simulink model "HaulagePhysicsKinematicsBridge"  (R2026a)
settings: Solver=ode23t  StopTime=390  MaxStep=0.05
PostLoadFcn:
  | stage12ModelFile = get_param(bdroot, 'FileName');
  | stage12ProjectRoot = fileparts(fileparts(stage12ModelFile));
  | addpath(stage12ProjectRoot);
  | loadStage12PhysicsKinematicsBridgeInputs(stage12ProjectRoot);
  | clear stage12ModelFile stage12ProjectRoot
InitFcn:
  | stage12ModelFile = get_param(bdroot, 'FileName');
  | stage12ProjectRoot = fileparts(fileparts(stage12ModelFile));
  | addpath(stage12ProjectRoot);
  | loadStage12PhysicsKinematicsBridgeInputs(stage12ProjectRoot);
  | clear stage12ModelFile stage12ProjectRoot
libraries: nesl_utility x6, fl_lib x3, sdl_lib x1, robotmobilelib x1
settings Model: Creator=chimb  LastModifiedBy=chimb

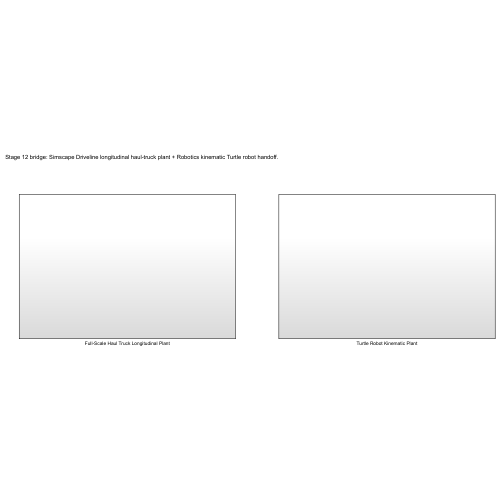
[thumbnail: Simulink's stored preview of the top-level diagram]
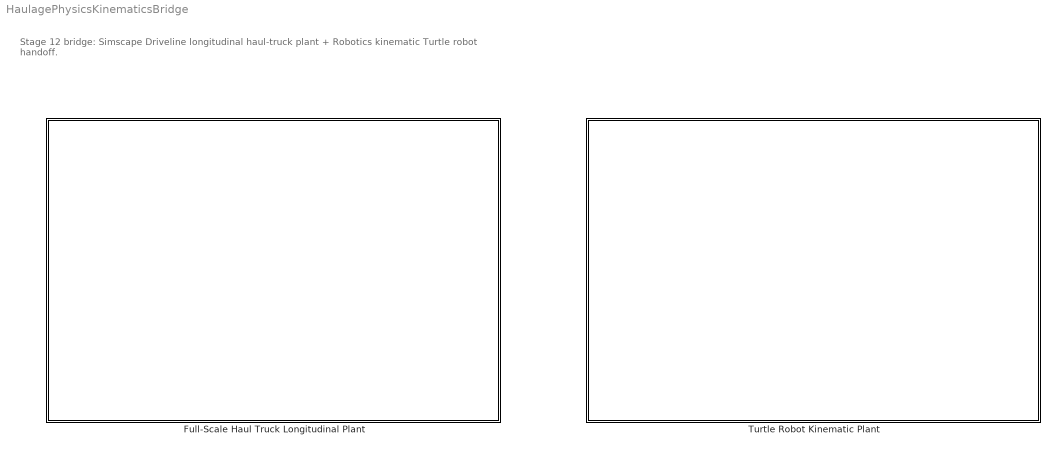
== system HaulagePhysicsKinematicsBridge ==
  note: Stage 12 bridge: Simscape Driveline longitudinal haul-truck plant + Robotics kinematic Turtle robot handoff.
  Full-Scale Haul Truck Longitudinal Plant : Subsystem
  Turtle Robot Kinematic Plant : Subsystem

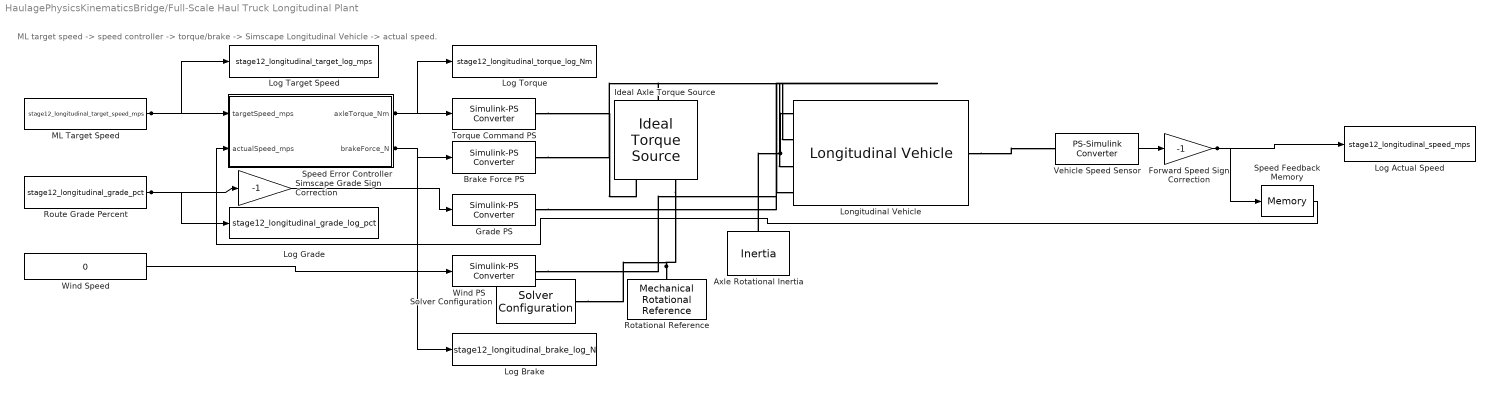
== system HaulagePhysicsKinematicsBridge/Full-Scale Haul Truck Longitudinal Plant ==
  note: ML target speed -> speed controller -> torque/brake -> Simscape Longitudinal Vehicle -> actual speed.
  Axle Rotational Inertia : fl_lib/Mechanical/Rotational Elements/Inertia  inertia=5000 kg*m^2  num_ports=foundation.enum.numPorts2.one  w_specify=off  w_priority=High  w=0 rad/s  w_nominal_specify=off  w_nominal_value=1  w_nominal_unit=rad/s  t_specify=off  t_priority=None  t=0 N*m  t_nominal_specify=off  t_nominal_value=1  t_nominal_unit=N*m
  Brake Force PS : nesl_utility/Simulink-PS Converter  PhysicalDomain=network_engine_domain  SubClassName=ps_input  LeftPortType=input  RightPortType=output  PseudoPeriodic=off  Frequencies=[]  NoiseDistribution=none  NoiseParameters=[]  Unit=1  AffineConversion=off  FilteringAndDerivatives=provide  SimscapeFilterOrder=1  InputFilterTimeConstant=0.001  UdotUserProvided=0
  Forward Speed Sign Correction : Gain  Gain=-1
  Grade PS : nesl_utility/Simulink-PS Converter  PhysicalDomain=network_engine_domain  SubClassName=ps_input  LeftPortType=input  RightPortType=output  PseudoPeriodic=off  Frequencies=[]  NoiseDistribution=none  NoiseParameters=[]  Unit=1  AffineConversion=off  FilteringAndDerivatives=provide  SimscapeFilterOrder=1  InputFilterTimeConstant=0.001  UdotUserProvided=0
  Ideal Axle Torque Source : fl_lib/Mechanical/Mechanical Sources/Ideal Torque Source
  Log Actual Speed : ToWorkspace  VariableName=stage12_longitudinal_speed_mps  SaveFormat=Timeseries  SampleTime=-1
  Log Brake : ToWorkspace  VariableName=stage12_longitudinal_brake_log_N  SaveFormat=Timeseries  SampleTime=-1
  Log Grade : ToWorkspace  VariableName=stage12_longitudinal_grade_log_pct  SaveFormat=Timeseries  SampleTime=-1
  Log Target Speed : ToWorkspace  VariableName=stage12_longitudinal_target_log_mps  SaveFormat=Timeseries  SampleTime=-1
  Log Torque : ToWorkspace  VariableName=stage12_longitudinal_torque_log_Nm  SaveFormat=Timeseries  SampleTime=-1
  Longitudinal Vehicle : sdl_lib/Tires & Vehicles/Longitudinal Vehicle  vehParamType=sdl.enum.VehicleParameterizationType.Regular  M_vehicle=429000 kg  R_tireroll=1.8 m  C_tireroll=0.03  C_airdrag=0.7  A_front=10 m^2  A_rl=120 N  B_rl=1.8 N*s/m  C_rl=0.389 N*s^2/m^2  g=9.81 m/s^2  V_1=0.3 m/s  w_1=0.01 rad/s  ShowBrakeIn=true  ShowSlopeIn=true  SlopeInputType=sdl.enum.VehicleLongitudinalRoadSlopeInputType.GradePercent  ShowWindIn=true  ShowGOut=false  air_density=1.184 kg/m^3  V_x_specify=off  V_x_priority=High  V_x=0 m/s  V_x_nominal_specify=off  V_x_nominal_value=1  V_x_nominal_unit=m/s  trq_specify=off  trq_priority=None  trq=0 N*m  trq_nominal_specify=off  trq_nominal_value=1  trq_nominal_unit=N*m  w_specify=off  w_priority=None  w=0 rad/s  w_nominal_specify=off  w_nominal_value=1  w_nominal_unit=rad/s
  ML Target Speed : FromWorkspace  VariableName=stage12_longitudinal_target_speed_mps
  Rotational Reference : fl_lib/Mechanical/Rotational Elements/Mechanical Rotational Reference
  Route Grade Percent : FromWorkspace  VariableName=stage12_longitudinal_grade_pct
  Simscape Grade Sign Correction : Gain  Gain=-1
  Solver Configuration : nesl_utility/Solver Configuration  PhysicalDomain=network_engine_domain  SubClassName=solver  LeftPortType=input  RightPortType=generic  Tones=[]  Harmonics=[]  SimulateNoise=off  Profile=off  UseLocalSampling=off  EnableSwitchedLinearOptims=on  FrequencyDomain=off  UseCCode=off  RelTol=0.001  AbsTol=0.001  MinStep=1e-09  ToWorkspace=off  RevertToSquareIcSolve=off  NumHomotopyIterations=100  PhasorMode=off  PhasorModeNumHarmonics=1  ConsistencySolver=NEWTON_XTOL_AFTER_FTOL  CanonicalOrdering=CANONICAL  OptimizeIntermediates=OPTIMIZED  IndexReductionMethod=DerivativeReplacement  DoDC=off  ResidualTolerance=1e-09  ConsistencyTolSource=GLOBAL  ConsistencyAbsTol=0.001  ConsistencyRelTol=0.001  ConsistencyTolFactor=0.001  UseLocalSolver=off  LocalSolverChoice=NE_BACKWARD_EULER_ADVANCER  ResolveIndetEquations=on  FunctionEvalNumThread=1  LocalSolverSampleTime=0.001  DoFixedCost=off  MaxNonlinIter=3  MaxModeIter=2  ComputeImpulses=off  ImpulseIterations=2  LinearAlgebra=auto  LinearAlgebraNumThread=0  EquationFormulation=NE_TIME_EF  DelaysMemoryBudget=1024  AutomaticFiltering=on  FilteringTimeConstant=0.001  PartitionStorageMethod=AS_NEEDED  PartitionMemoryBudget=1024  PartitionMethod=ROBUST  MultibodyUseLocalSolver=off  MultibodyLocalSolverChoice=ODE1  MultibodyLocalSolverSampleTime=0.001
  Speed Error Controller : MATLAB Function  TreatAsAtomicUnit=on
  Speed Feedback Memory : Memory
  Torque Command PS : nesl_utility/Simulink-PS Converter  PhysicalDomain=network_engine_domain  SubClassName=ps_input  LeftPortType=input  RightPortType=output  PseudoPeriodic=off  Frequencies=[]  NoiseDistribution=none  NoiseParameters=[]  Unit=1  AffineConversion=off  FilteringAndDerivatives=provide  SimscapeFilterOrder=1  InputFilterTimeConstant=0.001  UdotUserProvided=0
  Vehicle Speed Sensor : nesl_utility/PS-Simulink Converter  PhysicalDomain=network_engine_domain  SubClassName=ps_output  LeftPortType=input  RightPortType=output  PseudoPeriodic=off  Frequencies=[]  VectorFormat=inherit  Unit=inherit  AffineConversion=off
  Wind PS : nesl_utility/Simulink-PS Converter  PhysicalDomain=network_engine_domain  SubClassName=ps_input  LeftPortType=input  RightPortType=output  PseudoPeriodic=off  Frequencies=[]  NoiseDistribution=none  NoiseParameters=[]  Unit=1  AffineConversion=off  FilteringAndDerivatives=provide  SimscapeFilterOrder=1  InputFilterTimeConstant=0.001  UdotUserProvided=0
  Wind Speed : Constant  Value=0
  wires:
  ML Target Speed/1 -> Speed Error Controller/1(targetSpeed_mps), Log Target Speed/1
  Vehicle Speed Sensor/1 -> Forward Speed Sign Correction/1
  Forward Speed Sign Correction/1 -> Speed Feedback Memory/1, Log Actual Speed/1
  Speed Feedback Memory/1 -> Speed Error Controller/2(actualSpeed_mps)
  Speed Error Controller/1(axleTorque_Nm) -> Torque Command PS/1, Log Torque/1
  Speed Error Controller/2(brakeForce_N) -> Brake Force PS/1, Log Brake/1
  Route Grade Percent/1 -> Simscape Grade Sign Correction/1, Log Grade/1
  Simscape Grade Sign Correction/1 -> Grade PS/1
  Wind Speed/1 -> Wind PS/1
  connections:
  Torque Command PS/RConn1 -- Ideal Axle Torque Source/RConn1
  Longitudinal Vehicle/LConn1 -- Ideal Axle Torque Source/LConn1 -- Axle Rotational Inertia/LConn1
  Rotational Reference/LConn1 -- Ideal Axle Torque Source/RConn2 -- Solver Configuration/RConn1
  Brake Force PS/RConn1 -- Longitudinal Vehicle/LConn2
  Grade PS/RConn1 -- Longitudinal Vehicle/LConn3
  Wind PS/RConn1 -- Longitudinal Vehicle/LConn4
  Longitudinal Vehicle/RConn1 -- Vehicle Speed Sensor/LConn1

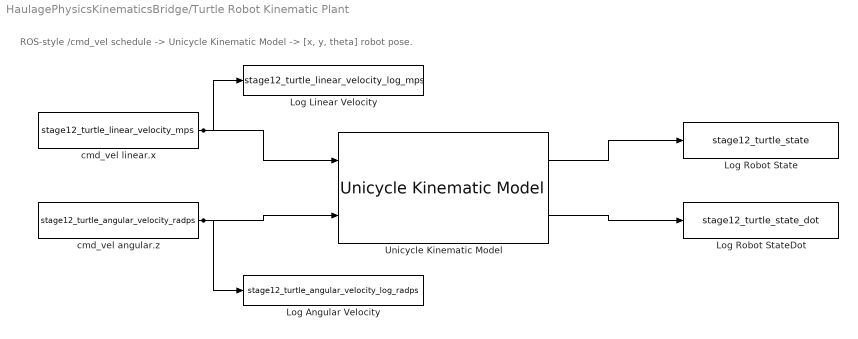
== system HaulagePhysicsKinematicsBridge/Turtle Robot Kinematic Plant ==
  note: ROS-style /cmd_vel schedule -> Unicycle Kinematic Model -> [x, y, theta] robot pose.
  Log Angular Velocity : ToWorkspace  VariableName=stage12_turtle_angular_velocity_log_radps  SaveFormat=Timeseries  SampleTime=-1
  Log Linear Velocity : ToWorkspace  VariableName=stage12_turtle_linear_velocity_log_mps  SaveFormat=Timeseries  SampleTime=-1
  Log Robot State : ToWorkspace  VariableName=stage12_turtle_state  SaveFormat=Timeseries  SampleTime=-1
  Log Robot StateDot : ToWorkspace  VariableName=stage12_turtle_state_dot  SaveFormat=Timeseries  SampleTime=-1
  Unicycle Kinematic Model : robotmobilelib/Unicycle Kinematic Model  VehicleInputs=Vehicle Speed & Heading Angular Velocity  WheelRadius=1.0  WheelSpeedRange=[0 0.3]  InitialState=[0; 0; 0]  SimulateUsing=Interpreted execution
  cmd_vel angular.z : FromWorkspace  VariableName=stage12_turtle_angular_velocity_radps  SampleTime=0.1  Interpolate=off  OutputAfterFinalValue=Setting to zero
  cmd_vel linear.x : FromWorkspace  VariableName=stage12_turtle_linear_velocity_mps  SampleTime=0.1  Interpolate=off  OutputAfterFinalValue=Setting to zero
  wires:
  cmd_vel linear.x/1 -> Unicycle Kinematic Model/1, Log Linear Velocity/1
  cmd_vel angular.z/1 -> Unicycle Kinematic Model/2, Log Angular Velocity/1
  Unicycle Kinematic Model/1 -> Log Robot State/1
  Unicycle Kinematic Model/2 -> Log Robot StateDot/1

== matlab function HaulagePhysicsKinematicsBridge/Full-Scale Haul Truck Longitudinal Plant/Speed Error Controller ==
  data: targetSpeed_mps input; axleTorque_Nm output; actualSpeed_mps input; brakeForce_N output
function [axleTorque_Nm, brakeForce_N] = f(targetSpeed_mps, actualSpeed_mps)
%#codegen
% Negative axle torque is the forward direction for this Simscape block orientation.
torqueGain = 120000;
brakeGain = 120000;
maxDriveTorque_Nm = 1100000;
maxBrakeForce_N = 300000;
speedError = targetSpeed_mps - actualSpeed_mps;
driveTorque = min(max(torqueGain * speedError, 0.0), maxDriveTorque_Nm);
brakeForce_N = 0.0;
axleTorque_Nm = -driveTorque;
end
